simulink library "Model_DG_CHP_Plant_Simscape"  (R2022b)
settings: Solver=VariableStepAuto  StartTime=0.0  StopTime=10.0  RelTol=1e-3
undefined symbols (not defined in the file): _cos_phi, _Q, _with_const_Q, a, b, c, d, P, V
libraries: ee_lib x11, nesl_utility x11, simulink x9, fl_lib x8, sps_avr x5, spsPositiveSequencePLLDrivenLib x3, eeGeneralControl x2, slpidlib x2, spsAC1AExcitationSystemLib x1, spsST2AExcitationSystemLib x1, Sublib_InternalFunctions x1, spsPLL3phLib x1
(part 1 of 2)
settings Model: Creator=winkens  LastModifiedBy=winkens
settings SolverCC: AlgebraicLoopSolver=TrustRegion
settings DebuggingCC: UnconnectedInputMsg=warning  UnconnectedOutputMsg=warning  UnconnectedLineMsg=warning  SFMachineParentedDataDiag=warning
settings ModelReferenceCC: EnableRefExpFcnMdlSchedulingChecks=on
settings RTWCC: DLArmComputeVersion=19.05

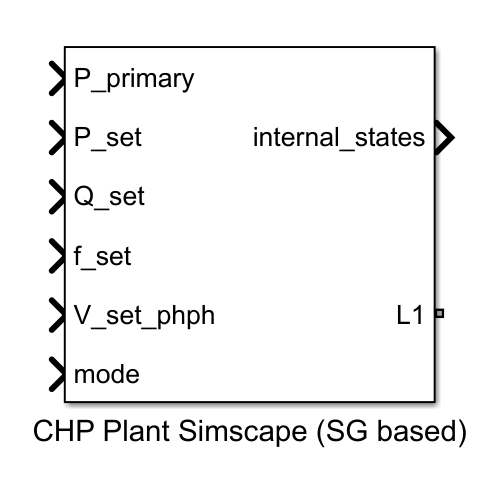
[thumbnail: Simulink's stored preview of the top-level diagram]
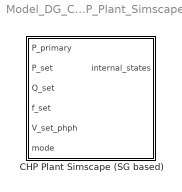
== system Model_DG_CHP_Plant_Simscape ==
  CHP Plant Simscape (SG based) : Subsystem  mask{S_n=3.2e6, V_n_phph=400, V_n_grid_phph=20e3, f_n=50, T_s=1e-4, nPolePairs=2, ReactancesSM=[3.19 0.33 0.159 1.79 0.155 0.05], X0=0.15, Ra=0.00074, TimeConstants=[0.5 0.025 0.025], K_IEEEG1simp=10, T_IEEEG1simp=[ 0.2 0 0.1 0 ], dP_maxmin_IEEEG1simp=[ 2 -2 ], exciterModel=AC1A, QCtrl=(d) Constant cos(phi), K_p_QCtrl=0.5, K_i_QCtrl=0.4, uq0ref=1.0, qmax=0.33, umax=1.04, deadband=0, p_pu=[0.1, 0.5, 0.6, 0.9, 1.0], q_pu=[0.0, 0.0, -0.05, -0.33, -0.33], p1=[0.94, 0.33], p2=[0.96, 0], p3=[1.04, 0], p4=[1.06, -0.33], cosphi_ref=1, ind_cap_Q=Inductive behavior (capacitive Q infeed), RL_Trafo_GenSide=[ 0.002 0.08 ], RL_Trafo_GridSide=[ 0.002 0.08 ], Rm=500, Lm=500, pu_X0=0.5}
      mask prompts: S_n "Nominal Apparent Power [VA]"; V_n_phph "Nominal Generator Voltage (rms, phase-to-phase) [V]"; V_n_grid_phph "Nominal Grid Voltage (rms, phase-to-phase) [V]"; f_n "Nominal Frequency [Hz]"; T_s "Sample Time [s]"; nPolePairs "Number of pole pairs"; ReactancesSM "Reactances Synchronous Machine [Xd Xd' Xd'' Xq Xq'' Xl] (pu)"; X0 "zero-sequence reactance X0 (pu)"; Ra "Stator Resistance Ra (pu)"; TimeConstants "Time Constants [Td' Td'' Tq''] (s)"; K_IEEEG1simp "Droop Gain dP/df (pu)"; T_IEEEG1simp "Time Constants [ T1 T2 T3 T4 ] (s)"; dP_maxmin_IEEEG1simp "Max. rate of change of mech. power [ dP_max dP_min ] (pu)"; exciterModel "Exciter Type"; QCtrl "Mode"; K_p_QCtrl "Q-Controller Proportional Gain"; K_i_QCtrl "Q-Controller Integral Gain"; uq0ref "U_Q0ref [pu]"; qmax "|Q_max| [pu]"; umax "U_max [pu]"; deadband "Voltage Deadband [+- %]"; p_pu "P_grid points [pu]"; q_pu "Q_grid points [pu]"; p1 "P1 [V_grid, Q_grid] [pu]"; p2 "P2 [V_grid, Q_grid] [pu]"; p3 "P3 [V_grid, Q_grid] [pu]"; p4 "P4 [V_grid, Q_grid] [pu]"; cosphi_ref "cos(phi)"; RL_Trafo_GenSide "Generator-Side-Impedance [ R L ] (pu):"; RL_Trafo_GridSide "Grid-Side-Impedance [ R L ] (pu):"; Rm "Magnetization resistance"; Lm "Magnetization inductance"; pu_X0 "zero sequence reactance"
      mask TypeOptions exciterModel: AC1A | AC4A | AC5A | DC1A | DC2A | ST1A | ST2A
      mask Callback exciterModel:
      | if strcmp(get_param(gcb,'exciterModel'),'AC1A')
      |     set_param([gcb '/SG_Control/Exciter'],'LabelModeActivechoice','AC1A');
      | 
      | elseif strcmp(get_param(gcb,'exciterModel'),'AC4A')
      |     set_param([gcb '/SG_Control/Exciter'],'LabelModeActivechoice','AC4A');
      | 
      | elseif strcmp(get_param(gcb,'exciterModel'),'AC5A')
      |     set_param([gcb '/SG_Control/Exciter'],'LabelModeActivechoice','AC5A');
      | 
      | elseif strcmp(get_param(gcb,'exciterModel'),'DC1A')
      |     set_param([gcb '/SG_Control/Exciter'],'LabelModeActivechoice','DC1A');
      | 
      | elseif strcmp(get_param(gcb,'exciterModel'),'DC2A')
      |     set_param([gcb '/SG_Control/Exciter'],'LabelModeActivechoice','DC2A');
      | 
      | elseif strcmp(get_param(gcb,'exciterModel'),'ST1A')
      |     set_param([gcb '/SG_Control/Exciter'],'LabelModeActivechoice','ST1A');
      | 
      | elseif strcmp(get_param(gcb,'exciterModel'),'ST2A')
      |     set_param([gcb '/SG_Control/Exciter'],'LabelModeActivechoice','ST2A');
      | 
      | else
      |     set_param([gcb '/SG_Control/Exciter'],'LabelModeActivechoice','DC1A');
      | 
      | end
      mask TypeOptions QCtrl: Constant Voltage (no Q-Control) | (a) Q(V)-Curve | (b) Q(P)-Curve | (c) Constant Q with Q(V)-Limitation | (d) Constant cos(phi)
      mask Callback QCtrl:
      | msk = Simulink.Mask.get(gcb);
      | if strcmp(get_param(gcb,'QCtrl'),'Constant Voltage (no Q-Control)')
      |     % no Q-Control
      |     msk.getDialogControl('paramboxVDE4110_Q_a').Visible = 'off';
      |     msk.getDialogControl('paramboxVDE4110_Q_b').Visible = 'off';
      |     msk.getDialogControl('paramboxVDE4110_Q_c').Visible = 'off';
      |     msk.getDialogControl('paramboxVDE4110_Q_d').Visible = 'off';
      |     set_param([gcb '/SG_Control/Reactive_Power_Controller'],'LabelModeActivechoice','const_V');
      | 
      | elseif strcmp(get_param(gcb,'QCtrl'),'(a) Q(V)-Curve')
      |     %(a) Q(V)
      |     msk.getDialogControl('paramboxVDE4110_Q_a').Visible = 'on';
      |     msk.getDialogControl('paramboxVDE4110_Q_b').Visible = 'off';
      |     msk.getDialogControl('paramboxVDE4110_Q_c').Visible = 'off';
      |     msk.getDialogControl('paramboxVDE4110_Q_d').Visible = 'off';
      |     set_param([gcb '/SG_Control/Reactive_Power_Controller'],'LabelModeActivechoice','(a)_Q(V)');
      | 
      | elseif strcmp(get_param(gcb,'QCtrl'),'(b) Q(P)-Curve')
      |     %(b) Q(P)
      |     msk.getDialogControl('paramboxVDE4110_Q_a').Visible = 'off';
      |     msk.getDialogControl('paramboxVDE4110_Q_b').Visible = 'on';
      |     msk.getDialogControl('paramboxVDE4110_Q_c').Visible = 'off';
      |     msk.getDialogControl('paramboxVDE4110_Q_d').Visible = 'off';
      |     set_param([gcb '/SG_Control/Reactive_Power_Controller'],'LabelModeActivechoice','(b)_Q(P)');
      | 
      | elseif strcmp(get_param(gcb,'QCtrl'),'(c) Constant Q with Q(V)-Limitation')
      |     %(c) const Q
      |     msk.getDialogControl('paramboxVDE4110_Q_a').Visible = 'off';
      |     msk.getDialogControl('paramboxVDE4110_Q_b').Visible = 'off';
      |     msk.getDialogControl('paramboxVDE4110_Q_c').Visible = 'on';
      |     msk.getDialogControl('paramboxVDE4110_Q_d').Visible = 'off';
      |     set_param([gcb '/SG_Control/Reactive_Power_Controller'],'LabelModeActivechoice','(c)_Q(V)_with_const_Q');
      | 
      | elseif strcmp(get_param(gcb,'QCtrl'),'(d) Constant cos(phi)')
      |     %(d) const cosphi
      |     msk.getDialogControl('paramboxVDE4110_Q_a').Visible = 'off';
      |     msk.getDialogControl('paramboxVDE4110_Q_b').Visible = 'off';
      |     msk.getDialogControl('paramboxVDE4110_Q_c').Visible = 'off';
      |     msk.getDialogControl('paramboxVDE4110_Q_d').Visible = 'on';
      |     set_param([gcb '/SG_Control/Reactive_Power_Controller'],'LabelModeActivechoice','(d)_cos_phi');
      | 
      | else
      |     % no Q-Control
      |     set_param([gcb '/SG_Control/Reactive_Power_Controller'],'LabelModeActivechoice','const_V');
      | 
      | end
      mask TypeOptions uq0ref: SG_Control/Reactive_Power_Controller/(a)_Q(V)/Q(V)_curve/uq0ref
      mask TypeOptions qmax: SG_Control/Reactive_Power_Controller/(a)_Q(V)/Q(V)_curve/qmax
      mask TypeOptions umax: SG_Control/Reactive_Power_Controller/(a)_Q(V)/Q(V)_curve/umax
      mask TypeOptions deadband: SG_Control/Reactive_Power_Controller/(a)_Q(V)/Q(V)_curve/deadband
      mask TypeOptions p_pu: SG_Control/Reactive_Power_Controller/(b)_Q(P)/Q(P)-curve/p_pu
      mask TypeOptions q_pu: SG_Control/Reactive_Power_Controller/(b)_Q(P)/Q(P)-curve/q_pu
      mask TypeOptions p1: SG_Control/Reactive_Power_Controller/(c)_Q(V)_with_const_Q/Q(V)_with_const_Q/p1
      mask TypeOptions p2: SG_Control/Reactive_Power_Controller/(c)_Q(V)_with_const_Q/Q(V)_with_const_Q/p2
      mask TypeOptions p3: SG_Control/Reactive_Power_Controller/(c)_Q(V)_with_const_Q/Q(V)_with_const_Q/p3
      mask TypeOptions p4: SG_Control/Reactive_Power_Controller/(c)_Q(V)_with_const_Q/Q(V)_with_const_Q/p4
      mask TypeOptions cosphi_ref: SG_Control/Reactive_Power_Controller/(d)_cos_phi/Constant_cos_phi/cosphi_ref
      mask TypeOptions ind_cap_Q: SG_Control/Reactive_Power_Controller/(d)_cos_phi/Constant_cos_phi/ind_cap_Q
      mask DialogControl DescGroupVar Prompt: CHP Plant (SG based)
      mask DialogControl DescTextVar Prompt: Combined-heat-and-power (CHP) plant using a synchronous generator (directly coupled to the grid) for electromechanical energy conversion.
      mask DialogControl Container4 Prompt: General
      mask DialogControl Container5 Prompt: Synchr. Gen.
      mask DialogControl Control2 Prompt: All Synchronous Generator Parameters are defined in a per-unit-system based on the nominal apparent power, nominal generator voltage and nominal frequency defined in general-tab.
      mask DialogControl Container11 Prompt: Parameters
      mask DialogControl Container6 Prompt: Governor
      mask DialogControl Container13 Prompt: Parameters (Simplified IEEEG1-Governor-Turbine-Model)
      mask DialogControl Container7 Prompt: Exciter
      mask DialogControl Container8 Prompt: Q-Control
      mask DialogControl Control3 Prompt: Quasi-steady state reactive power control based on German MV grid codes VDE4110. Choose constant voltage mode for no reactive power control.
      mask DialogControl Container17 Prompt: Parameters
      mask DialogControl paramboxVDE4110_Q_a Prompt: Q(V) Parameters
      mask DialogControl paramboxVDE4110_Q_b Prompt: Q(P) Parameters
      mask DialogControl paramboxVDE4110_Q_c Prompt: Constant Q with Q(V)-Limitation Parameters
      mask DialogControl paramboxVDE4110_Q_d Prompt: Constant cos(phi) Parameters
      mask DialogControl Container10 Prompt: Transformer
      mask DialogControl Control4 Prompt: Transformer parameters are defined in a per-unit-system based on the nominal power, the nominal frequency and the nominal voltages defined in tab General. The reference voltage for the impedance values depends on the respective nominal voltage level. However, magnetization resistance and inductance are based on the generator-side nominal voltage.
      mask DialogControl Container20 Prompt: Parameters

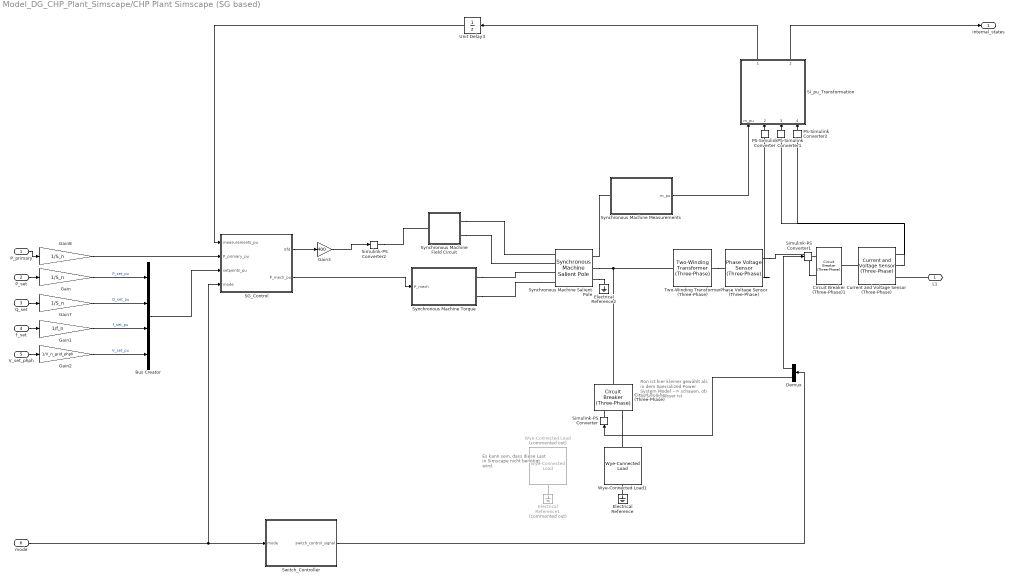
== system Model_DG_CHP_Plant_Simscape/CHP Plant Simscape (SG based) ==
  note: Ron ist hier kleiner gewählt als in dem Specialized Power System Model --> schauen, ob es so vllt besser ist
  note: Es kann sein, dass diese Last in Simscape nicht benötigt wird.
  P_primary : Inport
  P_set : Inport  Port=2
  Q_set : Inport  Port=3
  f_set : Inport  Port=4
  V_set_phph : Inport  Port=5
  mode : Inport  Port=6
  Bus Creator : BusCreator  Inputs=4
  Circuit Breaker (Three-Phase) : ee_lib/Switches & Breakers/Circuit Breaker (Three-Phase)  R_closed=0.001 Ohm  G_open=1e-6 1/Ohm  threshold=0.5 V  breaker_behavior=ee.enum.switches.breakerBehavior.zeroCrossingEnable
      settings: InternalSimscapePortConfiguration="{\"Bottom\":[],\"Left\":[{\"id\":\"vT\",\"label\":\"vT\",\"type\":\"input\"},{\"id\":\"N1\",\"label\":\"~1\",\"type\":\"foundation.electrical.three_phase\"}],\"Right\":[{\"id\":\"N2\",\"label\":\"~2\",\"type\":\"foundation.electrical.three_phase\"}],\"Top\":[]}"
  Circuit Breaker (Three-Phase)1 : ee_lib/Switches & Breakers/Circuit Breaker (Three-Phase)  R_closed=0.001 Ohm  G_open=1e-6 1/Ohm  threshold=0.5 V  breaker_behavior=ee.enum.switches.breakerBehavior.zeroCrossingEnable
      settings: InternalSimscapePortConfiguration="{\"Bottom\":[],\"Left\":[{\"id\":\"vT\",\"label\":\"vT\",\"type\":\"input\"},{\"id\":\"N1\",\"label\":\"~1\",\"type\":\"foundation.electrical.three_phase\"}],\"Right\":[{\"id\":\"N2\",\"label\":\"~2\",\"type\":\"foundation.electrical.three_phase\"}],\"Top\":[]}"
  Current and Voltage Sensor (Three-Phase) : ee_lib/Sensors & Transducers/Current and Voltage Sensor (Three-Phase)  vMeasurementType=ee.enum.vmeasurement.lg  outputUnit=ee.enum.unit.si  SRated=100e6 V*A  VRated=24e3 V  I_specify=off  I_priority=None  I=[ 0 0 0 ] A  I_nominal_specify=off  I_nominal_unit=A  I_nominal_value=1  V_specify=off  V_priority=None  V=[ 0 0 0 ] V  V_nominal_specify=off  V_nominal_unit=V  V_nominal_value=1
      settings: InternalSimscapePortConfiguration="{\"Bottom\":[],\"Left\":[{\"id\":\"N1\",\"label\":\"~1\",\"type\":\"foundation.electrical.three_phase\"}],\"Right\":[{\"id\":\"V_output\",\"label\":\"V\",\"type\":\"output\"},{\"id\":\"I_output\",\"label\":\"I\",\"type\":\"output\"},{\"id\":\"N2\",\"label\":\"~2\",\"type\":\"foundation.electrical.three_phase\"}],\"Top\":[]}"
  Demux : Demux  Outputs=2
  Electrical Reference : fl_lib/Electrical/Electrical Elements/Electrical Reference
  Electrical Reference1 : fl_lib/Electrical/Electrical Elements/Electrical Reference  Commented=on
  Electrical Reference2 : fl_lib/Electrical/Electrical Elements/Electrical Reference
  Gain : Gain  Gain=1/S_n
  Gain1 : Gain  Gain=1/f_n
  Gain2 : Gain  Gain=1/V_n_grid_phph
  Gain3 : Gain  Gain=400
  Gain7 : Gain  Gain=1/S_n
  Gain8 : Gain  Gain=1/S_n
  PS-Simulink Converter : nesl_utility/PS-Simulink Converter  PhysicalDomain=network_engine_domain  SubClassName=ps_output  LeftPortType=input  RightPortType=output  PseudoPeriodic=off  Frequencies=[]  VectorFormat=1-D array  Unit=inherit  AffineConversion=off
  PS-Simulink Converter1 : nesl_utility/PS-Simulink Converter  PhysicalDomain=network_engine_domain  SubClassName=ps_output  LeftPortType=input  RightPortType=output  PseudoPeriodic=off  Frequencies=[]  VectorFormat=1-D array  Unit=inherit  AffineConversion=off
  PS-Simulink Converter2 : nesl_utility/PS-Simulink Converter  PhysicalDomain=network_engine_domain  SubClassName=ps_output  LeftPortType=input  RightPortType=output  PseudoPeriodic=off  Frequencies=[]  VectorFormat=1-D array  Unit=inherit  AffineConversion=off
  Phase Voltage Sensor (Three-Phase) : ee_lib/Sensors & Transducers/Phase Voltage Sensor (Three-Phase)
  SG_Control : Subsystem
  SI_pu_Transformation : Subsystem
  Simulink-PS Converter : nesl_utility/Simulink-PS Converter  PhysicalDomain=network_engine_domain  SubClassName=ps_input  LeftPortType=input  RightPortType=output  PseudoPeriodic=off  Frequencies=[]  NoiseDistribution=none  NoiseParameters=[]  Unit=1  AffineConversion=off  FilteringAndDerivatives=provide  SimscapeFilterOrder=1  InputFilterTimeConstant=0.001  UdotUserProvided=0
  Simulink-PS Converter1 : nesl_utility/Simulink-PS Converter  PhysicalDomain=network_engine_domain  SubClassName=ps_input  LeftPortType=input  RightPortType=output  PseudoPeriodic=off  Frequencies=[]  NoiseDistribution=none  NoiseParameters=[]  Unit=1  AffineConversion=off  FilteringAndDerivatives=provide  SimscapeFilterOrder=1  InputFilterTimeConstant=0.001  UdotUserProvided=0
  Simulink-PS Converter2 : nesl_utility/Simulink-PS Converter  PhysicalDomain=network_engine_domain  SubClassName=ps_input  LeftPortType=input  RightPortType=output  PseudoPeriodic=off  Frequencies=[]  NoiseDistribution=none  NoiseParameters=[]  Unit=1  AffineConversion=off  FilteringAndDerivatives=provide  SimscapeFilterOrder=1  InputFilterTimeConstant=0.001  UdotUserProvided=0
  Switch_Controller : Subsystem
  Synchronous Machine Salient Pole : ee_lib/Electromechanical/Synchronous/Synchronous Machine Salient Pole  port_option=ee.enum.threePhasePort.composite  SRated=S_n V*A  VRated=V_n_phph V  FRated=f_n Hz  nPolePairs=2  param_option=ee.enum.sm.parameterization.standard  fieldCircuitParameterization_option=ee.enum.sm.fieldparameterization.current  baseEfd=400 V  baseIfd=22 A  zero_sequence=ee.enum.park.zerosequence.include  axes_param=ee.enum.rotorangle.daxis  Ladu=0.9  Laqu=0.55  L0=0.15  Ll=0.15  Ra=Ra  Lfd=0.2571  Rfd=0.0006  L1d=0.2  R1d=0.0354  L1q=0.2567  R1q=0.0428  Xl=ReactancesSM(6)  Xd=ReactancesSM(1)  Xq=ReactancesSM(4)  X0=X0  Xdd=ReactancesSM(2)  Xddd=ReactancesSM(3)  Xqdd=ReactancesSM(5)  d_option=ee.enum.circuit.short  Td0d=5.25 s  Tdd=TimeConstants(1) s  Td0dd=0.03 s  Tddd=TimeConstants(2) s  q_option=ee.enum.circuit.short  Tq0dd=0.05 s  Tqdd=TimeConstants(3) s  saturation_option=ee.enum.saturation.exclude  saturation_ifd=[0, .48, .76, 1.38, 1.79]  saturation_Vag=[0, .43, .59, .71, .76]  initialization_option=ee.enum.sm.initialization.electrical  source_type=ee.enum.sm.load_flow_source_type.Swing  Vmag0=V_n_phph V  Vang0=0 deg  Pt0=1.2e6 V*A  Qt0=0.4e6 V*A  minimum_pu=0.95  phase_search_range=[-30, 30] deg  gmin=0 S  connection_option=ee.enum.Connection.wye  num_q_dampers=1  rotor_offset=-pi / 2 rad  pu_psid_specify=on  pu_psid_priority=High  pu_psid=0  pu_psid_nominal_specify=off  pu_psid_nominal_unit=1  pu_psid_nominal_value=1  pu_psiq_specify=on  pu_psiq_priority=High  pu_psiq=0  pu_psiq_nominal_specify=off  pu_psiq_nominal_unit=1  pu_psiq_nominal_value=1  pu_psifd_specify=on  pu_psifd_priority=High  pu_psifd=0  pu_psifd_nominal_specify=off  pu_psifd_nominal_unit=1  pu_psifd_nominal_value=1  pu_psi1d_specify=on  pu_psi1d_priority=High  pu_psi1d=0  pu_psi1d_nominal_specify=off  pu_psi1d_nominal_unit=1  pu_psi1d_nominal_value=1  pu_psi1q_specify=on  pu_psi1q_priority=High  pu_psi1q=0  pu_psi1q_nominal_specify=off  pu_psi1q_nominal_unit=1  pu_psi1q_nominal_value=1  angular_position_diff_specify=on  angular_position_diff_priority=High  angular_position_diff=-pi/2/nPolePairs rad  angular_position_diff_nominal_specify=off  angular_position_diff_nominal_unit=deg  angular_position_diff_nominal_value=1  Tmeas=298.15 K  alpha=3.93e-3 1/K  stator_thermal_mass=100 J/K  rotor_thermal_mass=200 J/K  temperatureA_specify=off  temperatureA_priority=High  temperatureA=25 degC  temperatureA_nominal_specify=off  temperatureA_nominal_unit=degC  temperatureA_nominal_value=1  temperatureB_specify=off  temperatureB_priority=High  temperatureB=25 degC  temperatureB_nominal_specify=off  temperatureB_nominal_unit=degC  temperatureB_nominal_value=1  temperatureC_specify=off  temperatureC_priority=High  temperatureC=25 degC  temperatureC_nominal_specify=off  temperatureC_nominal_unit=degC  temperatureC_nominal_value=1  temperatureR_specify=off  temperatureR_priority=High  temperatureR=25 degC  temperatureR_nominal_specify=off  temperatureR_nominal_unit=degC  temperatureR_nominal_value=1
      settings: InternalSimscapePortConfiguration="{\"Bottom\":[],\"Left\":[{\"id\":\"fd_p\",\"label\":\"fd+\",\"type\":\"foundation.electrical.electrical\"},{\"id\":\"fd_n\",\"label\":\"fd-\",\"type\":\"foundation.electrical.electrical\"},{\"id\":\"R\",\"label\":\"R\",\"type\":\"foundation.mechanical.rotational.rotational\"},{\"id\":\"C\",\"label\":\"C\",\"type\":\"foundation.mechanical.rotational.rotational\"}],\"Right\":[{\"id\":\"pu_output\",\"label\":\"pu\",\"type\":\"output\"},{\"id\":\"N\",\"label\":\"~\",\"type\":\"foundation.electrical.three_phase\"},{\"id\":\"n\",\"label\":\"n\",\"type\":\"foundation.electrical.electrical\"}],\"Top\":[]}"
  Synchronous Machine Field Circuit : Subsystem
  Synchronous Machine Measurements : Subsystem
  Synchronous Machine Torque : Subsystem
  Two-Winding Transformer (Three-Phase) : ee_lib/Passive/Transformers/Two-Winding Transformer (Three-Phase)  SRated=S_n V*A  FRated=f_n Hz  Winding1Connection=ee.enum.windingconnection.Yg  VRated1=V_n_phph V  Winding2Connection=ee.enum.windingconnection.delta11  VRated2=V_n_grid_phph V  CoreType=ee.enum.coretype.threelimb  pu_Rw1=RL_Trafo_GenSide(1)  pu_Rw2=RL_Trafo_GridSide(1)  leakage_reactance_option=ee.enum.transformer_leakage.include  pu_Xl1=RL_Trafo_GenSide(2)  pu_Xl2=RL_Trafo_GridSide(2)  magnetizing_resistance_option=ee.enum.transformer_magnetizingResistance.include  pu_Rm=Rm  magnetizing_reactance_option=ee.enum.transformer_magnetizingReactance.include  saturation_option=ee.enum.transformer_saturation.exclude  pu_Xm=Lm  current_data=[0, .002, 1, 2]  magnetic_flux_data=[0, 1.2, 1.5, 1.51]  pu_X0=pu_X0  i1_specify=off  i1_priority=None  i1=[ 0 0 0 ] A  i1_nominal_specify=off  i1_nominal_unit=A  i1_nominal_value=1  i2_specify=off  i2_priority=None  i2=[ 0 0 0 ] A  i2_nominal_specify=off  i2_nominal_unit=A  i2_nominal_value=1  phi_specify=off  phi_priority=None  phi=[ 0 0 0 ]  phi_nominal_specify=off  phi_nominal_unit=1  phi_nominal_value=1  power_dissipated_specify=off  power_dissipated_priority=None  power_dissipated=0 W  power_dissipated_nominal_specify=off  power_dissipated_nominal_unit=W  power_dissipated_nominal_value=1
      settings: InternalSimscapePortConfiguration="{\"Bottom\":[],\"Left\":[{\"id\":\"N1\",\"label\":\"~1\",\"type\":\"foundation.electrical.three_phase\"}],\"Right\":[{\"id\":\"N2\",\"label\":\"~2\",\"type\":\"foundation.electrical.three_phase\"}],\"Top\":[]}"
  Unit Delay3 : UnitDelay  SampleTime=-1  HasFrameUpgradeWarning=on
  Wye-Connected Load : ee_lib/Passive/RLC Assemblies/Wye-Connected Load  Commented=on  parameterization=2  component_structure=1  component_structure_PQ=1  R=1 Ohm  L=1e-3 H  C=1e-6 F  VRated=V_n_phph V  FRated=60 Hz  P=0.001*S_n W  Qpos=1e2 V*A  Qneg=-1e2 V*A  R_parasitic=1e-6 Ohm  G_parasitic=1e-6 1/Ohm  R_parasitic_PQ=1e-6 Ohm  G_parasitic_PQ=1e-6 1/Ohm  Vmag0=24e3 V  Vang0=0 deg  Freq0=60 Hz  IL_specify=on  IL_priority=High  IL=[0, 0, 0] A  IL_nominal_specify=off  IL_nominal_unit=A  IL_nominal_value=1  VC_specify=on  VC_priority=High  VC=[0, 0, 0] V  VC_nominal_specify=off  VC_nominal_unit=V  VC_nominal_value=1
  Wye-Connected Load1 : ee_lib/Passive/RLC Assemblies/Wye-Connected Load  parameterization=2  component_structure=1  component_structure_PQ=1  R=1 Ohm  L=1e-3 H  C=1e-6 F  VRated=V_n_phph V  FRated=60 Hz  P=0.2*S_n W  Qpos=1e2 V*A  Qneg=-1e2 V*A  R_parasitic=1e-6 Ohm  G_parasitic=1e-6 1/Ohm  R_parasitic_PQ=1e-6 Ohm  G_parasitic_PQ=1e-6 1/Ohm  Vmag0=24e3 V  Vang0=0 deg  Freq0=60 Hz  IL_specify=on  IL_priority=High  IL=[0, 0, 0] A  IL_nominal_specify=off  IL_nominal_unit=A  IL_nominal_value=1  VC_specify=on  VC_priority=High  VC=[0, 0, 0] V  VC_nominal_specify=off  VC_nominal_unit=V  VC_nominal_value=1
  L1 : PMIOPort  Side=Right
  internal_states : Outport
  wires:
  V_set_phph/1 -> Gain2/1
  P_set/1 -> Gain/1
  f_set/1 -> Gain1/1
  SI_pu_Transformation/2(measurements_SI) -> internal_states/1
  SI_pu_Transformation/1(measurements_pu) -> Unit Delay3/1
  Q_set/1 -> Gain7/1
  P_primary/1 -> Gain8/1
  Gain/1 -> Bus Creator/1  "P_set_pu"
  Gain7/1 -> Bus Creator/2  "Q_set_pu"
  Gain1/1 -> Bus Creator/3  "f_set_pu"
  Gain2/1 -> Bus Creator/4  "V_set_pu"
  Switch_Controller/1(switch_control_signal) -> Demux/1
  Demux/2 -> Simulink-PS Converter/1
  PS-Simulink Converter/1 -> SI_pu_Transformation/2(V_breaker_SI)
  Demux/1 -> Simulink-PS Converter1/1
  PS-Simulink Converter1/1 -> SI_pu_Transformation/3(V_grid_SI)
  PS-Simulink Converter2/1 -> SI_pu_Transformation/4(I_grid_SI)
  Gain8/1 -> SG_Control/2(P_primary_pu)
  mode/1 -> SG_Control/4(mode), Switch_Controller/1(mode)
  Bus Creator/1 -> SG_Control/3(setpoints_pu)
  Unit Delay3/1 -> SG_Control/1(measurements_pu)
  Synchronous Machine Measurements/1(m_pu) -> SI_pu_Transformation/1(m_pu)
  SG_Control/2(P_mech_pu) -> Synchronous Machine Torque/1(P_mech)
  Gain3/1 -> Simulink-PS Converter2/1
  SG_Control/1(Efd) -> Gain3/1
  connections:
  Synchronous Machine Salient Pole/RConn2 -- Two-Winding Transformer (Three-Phase)/LConn1 -- Circuit Breaker (Three-Phase)/RConn1
  Circuit Breaker (Three-Phase)/LConn2 -- Wye-Connected Load1/LConn1
  Simulink-PS Converter/RConn1 -- Circuit Breaker (Three-Phase)/LConn1
  Electrical Reference/LConn1 -- Wye-Connected Load1/RConn1
  Electrical Reference1/LConn1 -- Wye-Connected Load/RConn1
  Two-Winding Transformer (Three-Phase)/RConn1 -- Phase Voltage Sensor (Three-Phase)/LConn1
  Phase Voltage Sensor (Three-Phase)/RConn1 -- PS-Simulink Converter/LConn1
  Phase Voltage Sensor (Three-Phase)/RConn2 -- Circuit Breaker (Three-Phase)1/LConn2
  Simulink-PS Converter1/RConn1 -- Circuit Breaker (Three-Phase)1/LConn1
  Current and Voltage Sensor (Three-Phase)/LConn1 -- Circuit Breaker (Three-Phase)1/RConn1
  Current and Voltage Sensor (Three-Phase)/RConn2 -- PS-Simulink Converter2/LConn1
  L1/RConn1 -- Current and Voltage Sensor (Three-Phase)/RConn3
  Synchronous Machine Salient Pole/RConn3 -- Electrical Reference2/LConn1
  PS-Simulink Converter1/LConn1 -- Current and Voltage Sensor (Three-Phase)/RConn1
  Simulink-PS Converter2/RConn1 -- Synchronous Machine Field Circuit/LConn1
  Synchronous Machine Field Circuit/RConn1 -- Synchronous Machine Salient Pole/LConn1
  Synchronous Machine Field Circuit/RConn2 -- Synchronous Machine Salient Pole/LConn2
  Synchronous Machine Salient Pole/RConn1 -- Synchronous Machine Measurements/LConn1
  Synchronous Machine Torque/RConn1 -- Synchronous Machine Salient Pole/LConn3
  Synchronous Machine Torque/RConn2 -- Synchronous Machine Salient Pole/LConn4

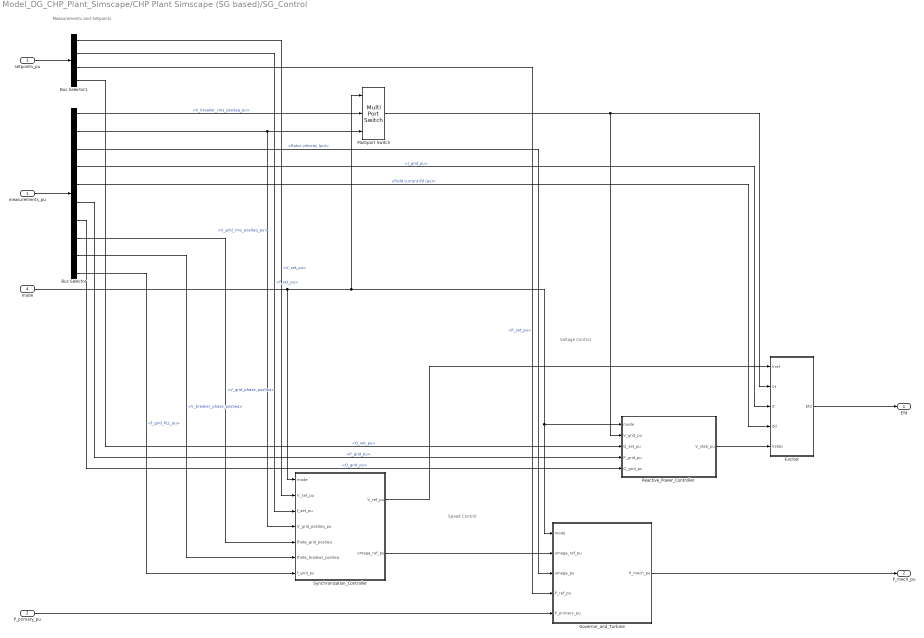
== system Model_DG_CHP_Plant_Simscape/CHP Plant Simscape (SG based)/SG_Control ==
  note: Speed Control
  note: Voltage Control
  note: Measurements and Setpoints
  measurements_pu : Inport
  P_primary_pu : Inport  Port=2
  setpoints_pu : Inport  Port=3
  mode : Inport  Port=4
  Bus Selector : BusSelector  OutputSignals=electrical_pu.V_breaker_rms_posSeq_pu,electrical_pu.V_grid_rms_posSeq_pu,SG_pu.Rotor velocity (pu),electrical_pu.I_grid_pu,SG_pu.Field current Ifd (pu),electrical_pu.P_grid_pu,electrical_pu.Q_grid_pu,electrical_pu.V_grid_phase_posSeq,electrical_pu.V_breaker_phase_posSeq,electrical_pu.f_grid_PLL_pu
  Bus Selector1 : BusSelector  OutputSignals=V_set_pu,f_set_pu,P_set_pu,Q_set_pu
  Exciter : Subsystem  Variant=on  VariantControlMode=label  LabelModeActiveChoice=AC1A
      settings: AttributesFormatString=%<BlockChoice>
  Governor_and_Turbine : Subsystem  Variant=on  VariantControlMode=label  LabelModeActiveChoice=IEEEG1_simplified
  Multiport Switch : MultiPortSwitch  Inputs=2  DiagnosticForDefault=None  SaturateOnIntegerOverflow=off  InputSameDT=off
  Reactive_Power_Controller : Subsystem  Variant=on  VariantControlMode=label  LabelModeActiveChoice=(d)_cos_phi
  Synchronization_Controller : Subsystem
  Efd : Outport
  P_mech_pu : Outport  Port=2
  wires:
  Exciter/1(Efd) -> Efd/1
  Governor_and_Turbine/1(P_mech_pu) -> P_mech_pu/1
  Reactive_Power_Controller/1(V_stab_pu) -> Exciter/5(Vstab)
  measurements_pu/1 -> Bus Selector/1
  setpoints_pu/1 -> Bus Selector1/1
  Bus Selector1/3 -> Governor_and_Turbine/4(P_ref_pu)  "<P_set_pu>"
  Bus Selector/3 -> Governor_and_Turbine/3(omega_pu)  "<Rotor velocity (pu)>"
  P_primary_pu/1 -> Governor_and_Turbine/5(P_primary_pu)
  Multiport Switch/1 -> Reactive_Power_Controller/2(V_grid_pu), Exciter/2(Vt)
  Bus Selector/4 -> Exciter/3(It)  "<I_grid_pu>"
  Bus Selector/5 -> Exciter/4(Ifd)  "<Field current Ifd (pu)>"
  mode/1 -> Multiport Switch/1, Governor_and_Turbine/1(mode), Reactive_Power_Controller/1(mode), Synchronization_Controller/1(mode)
  Bus Selector1/4 -> Reactive_Power_Controller/3(Q_set_pu)  "<Q_set_pu>"
  Bus Selector/2 -> Synchronization_Controller/4(V_grid_posSeq_pu), Multiport Switch/3  "<V_grid_rms_posSeq_pu>"
  Bus Selector/1 -> Multiport Switch/2  "<V_breaker_rms_posSeq_pu>"
  Bus Selector/6 -> Reactive_Power_Controller/4(P_grid_pu)  "<P_grid_pu>"
  Bus Selector/7 -> Reactive_Power_Controller/5(Q_grid_pu)  "<Q_grid_pu>"
  Synchronization_Controller/2(omega_ref_pu) -> Governor_and_Turbine/2(omega_ref_pu)
  Synchronization_Controller/1(V_ref_pu) -> Exciter/1(Vref)
  Bus Selector1/1 -> Synchronization_Controller/2(V_set_pu)  "<V_set_pu>"
  Bus Selector1/2 -> Synchronization_Controller/3(f_set_pu)  "<f_set_pu>"
  Bus Selector/8 -> Synchronization_Controller/5(theta_grid_posSeq)  "<V_grid_phase_posSeq>"
  Bus Selector/9 -> Synchronization_Controller/6(theta_breaker_posSeq)  "<V_breaker_phase_posSeq>"
  Bus Selector/10 -> Synchronization_Controller/7(f_grid_pu)  "<f_grid_PLL_pu>"

== system Model_DG_CHP_Plant_Simscape/CHP Plant Simscape (SG based)/SI_pu_Transformation ==
  m_pu : Inport
  V_breaker_SI : Inport  Port=2
  V_grid_SI : Inport  Port=3
  I_grid_SI : Inport  Port=4
  Bus Creator : BusCreator  Inputs=11
  Bus Creator1 : BusCreator  Inputs=2
  Bus Creator2 : BusCreator  Inputs=2
  Electrical_Measurements_To_pu : Subsystem
  Positive_Sequence_Calculation : Subsystem
  SG_Measurements_To_SI : Subsystem
  measurements_pu : Outport
  measurements_SI : Outport  Port=2
  wires:
  m_pu/1 -> Bus Creator2/1, SG_Measurements_To_SI/1(m_pu)  "SG_pu"
  V_breaker_SI/1 -> Positive_Sequence_Calculation/2(V_breaker_abc), Bus Creator/1  "V_breaker_SI"
  V_grid_SI/1 -> Positive_Sequence_Calculation/1(V_grid_abc), Bus Creator/2  "V_grid_SI"
  I_grid_SI/1 -> Positive_Sequence_Calculation/3(I_grid_abc), Bus Creator/3  "I_grid_SI"
  Bus Creator/1 -> Bus Creator1/2, Electrical_Measurements_To_pu/1(el_SI)  "electrical_SI"
  Bus Creator1/1 -> measurements_SI/1
  Bus Creator2/1 -> measurements_pu/1
  Electrical_Measurements_To_pu/1(el_pu) -> Bus Creator2/2  "electrical_pu"
  SG_Measurements_To_SI/1(m_SI) -> Bus Creator1/1  "SG_SI"
  Positive_Sequence_Calculation/1(P_grid_SI) -> Bus Creator/4  "P_grid_SI"
  Positive_Sequence_Calculation/2(Q_grid_SI) -> Bus Creator/5  "Q_grid_SI"
  Positive_Sequence_Calculation/3(V_grid_rms_posSeq_SI) -> Bus Creator/6  "V_grid_rms_posSeq_SI"
  Positive_Sequence_Calculation/4(I_grid_rms_posSeq_SI) -> Bus Creator/7  "I_grid_rms_posSeq_SI"
  Positive_Sequence_Calculation/5(V_breaker_rms_posSeq_SI) -> Bus Creator/8  "V_breaker_rms_posSeq_SI"
  Positive_Sequence_Calculation/6(V_grid_phase_posSeq_SI) -> Bus Creator/9  "V_grid_phase_posSeq"
  Positive_Sequence_Calculation/7(V_breaker_phase_posSeq_SI) -> Bus Creator/10  "V_breaker_phase_posSeq"
  Positive_Sequence_Calculation/8(f_grid_PLL_SI) -> Bus Creator/11  "f_grid_PLL_SI"

== system Model_DG_CHP_Plant_Simscape/CHP Plant Simscape (SG based)/Switch_Controller ==
  note: Blackstart
  note: Synchronization
  note: Grid Parallel Operation
  mode : Inport
  Constant{,1..3} (4 alike) : Constant  Value=0
  Constant4 : Constant
  Constant5 : Constant
  Multiport Switch : MultiPortSwitch  DataPortOrder=Zero-based contiguous  zeroidx=on  SaturateOnIntegerOverflow=off  InputSameDT=off
  Mux : Mux  Inputs=2
  Mux1 : Mux  Inputs=2
  Mux2 : Mux  Inputs=2
  switch_control_signal : Outport
  wires:
  mode/1 -> Multiport Switch/1
  Multiport Switch/1 -> switch_control_signal/1
  Mux/1 -> Multiport Switch/2
  Mux2/1 -> Multiport Switch/4
  Mux1/1 -> Multiport Switch/3
  Constant/1 -> Mux/1
  Constant1/1 -> Mux/2
  Constant2/1 -> Mux2/1
  Constant3/1 -> Mux1/2
  Constant4/1 -> Mux1/1
  Constant5/1 -> Mux2/2

== system Model_DG_CHP_Plant_Simscape/CHP Plant Simscape (SG based)/Synchronous Machine Field Circuit ==
  Controlled Voltage Source : fl_lib/Electrical/Electrical Sources/Controlled Voltage Source
  Electrical Reference2 : fl_lib/Electrical/Electrical Elements/Electrical Reference
  Efd : PMIOPort  Side=Left
  fd+ : PMIOPort  Port=2  Side=Right
  fd- : PMIOPort  Port=3  Side=Right
  connections:
  Efd/RConn1 -- Controlled Voltage Source/RConn1
  Controlled Voltage Source/LConn1 -- fd+/RConn1
  Controlled Voltage Source/RConn2 -- Electrical Reference2/LConn1 -- fd-/RConn1

== system Model_DG_CHP_Plant_Simscape/CHP Plant Simscape (SG based)/Synchronous Machine Measurements ==
  Bus Creator1 : BusCreator  Inputs=2
  PS-Simulink Converter4 : nesl_utility/PS-Simulink Converter  PhysicalDomain=network_engine_domain  SubClassName=ps_output  LeftPortType=input  RightPortType=output  PseudoPeriodic=off  Frequencies=[]  VectorFormat=1-D array  Unit=inherit  AffineConversion=off
  PS-Simulink Converter5 : nesl_utility/PS-Simulink Converter  PhysicalDomain=network_engine_domain  SubClassName=ps_output  LeftPortType=input  RightPortType=output  PseudoPeriodic=off  Frequencies=[]  VectorFormat=1-D array  Unit=inherit  AffineConversion=off
  Synchronous Machine Measurement : ee_lib/Electromechanical/Synchronous/Synchronous Machine Measurement  output_idx=2
      settings: InternalSimscapePortConfiguration="{\"Bottom\":[],\"Left\":[{\"id\":\"pu_input\",\"label\":\"pu\",\"type\":\"input\"}],\"Right\":[{\"id\":\"pu_output\",\"label\":\"o\",\"type\":\"output\"}],\"Top\":[]}"
  Synchronous Machine Measurement1 : ee_lib/Electromechanical/Synchronous/Synchronous Machine Measurement  output_idx=4
      settings: InternalSimscapePortConfiguration="{\"Bottom\":[],\"Left\":[{\"id\":\"pu_input\",\"label\":\"pu\",\"type\":\"input\"}],\"Right\":[{\"id\":\"pu_output\",\"label\":\"o\",\"type\":\"output\"}],\"Top\":[]}"
  pu : PMIOPort  Side=Left
  m_pu : Outport
  wires:
  PS-Simulink Converter4/1 -> Bus Creator1/1  "Field current Ifd (pu)"
  PS-Simulink Converter5/1 -> Bus Creator1/2  "Rotor velocity (pu)"
  Bus Creator1/1 -> m_pu/1
  connections:
  Synchronous Machine Measurement/LConn1 -- Synchronous Machine Measurement1/LConn1 -- pu/RConn1
  Synchronous Machine Measurement/RConn1 -- PS-Simulink Converter4/LConn1
  Synchronous Machine Measurement1/RConn1 -- PS-Simulink Converter5/LConn1

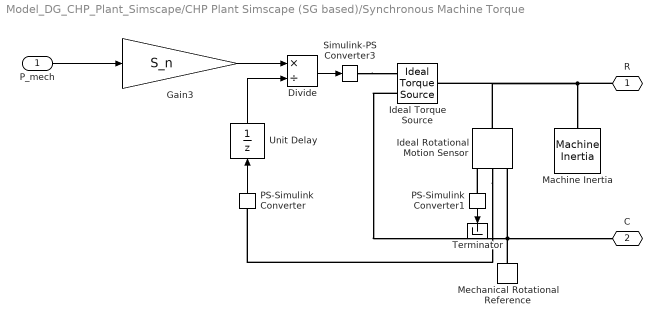
== system Model_DG_CHP_Plant_Simscape/CHP Plant Simscape (SG based)/Synchronous Machine Torque ==
  P_mech : Inport
  Divide : Product  Inputs=*/
  Gain3 : Gain  Gain=S_n
  Ideal Rotational Motion Sensor : fl_lib/Mechanical/Mechanical Sensors/Ideal Rotational Motion Sensor  reference=foundation.enum.MeasurementReference.difference  acceleration_port=false  velocity_port=true  position_port=true  wrap_angle=simscape.enum.onoff.off  offset=0 rad
  Ideal Torque Source : fl_lib/Mechanical/Mechanical Sources/Ideal Torque Source
  Machine Inertia : ee_lib/Electromechanical/Mechanical/Machine Inertia  SRated=S_n V*A  FRated=f_n Hz  nPolePairs=nPolePairs  inertia_option=2  J=27548 kg*m^2  H=0.02 s*W/V/A  damper_option=2  D=39.0509 N*m/(rad/s)  pu_D=0.01  initialization_option=2  fMechanical0=60 Hz  fElectrical0=f_n Hz
      settings: InternalSimscapePortConfiguration="{\"Bottom\":[],\"Left\":[{\"id\":\"R\",\"label\":\"R\",\"type\":\"foundation.mechanical.rotational.rotational\"}],\"Right\":[],\"Top\":[]}"
  Mechanical Rotational Reference : fl_lib/Mechanical/Rotational Elements/Mechanical Rotational Reference
  PS-Simulink Converter : nesl_utility/PS-Simulink Converter  PhysicalDomain=network_engine_domain  SubClassName=ps_output  LeftPortType=input  RightPortType=output  PseudoPeriodic=off  Frequencies=[]  VectorFormat=1-D array  Unit=inherit  AffineConversion=off
  PS-Simulink Converter1 : nesl_utility/PS-Simulink Converter  PhysicalDomain=network_engine_domain  SubClassName=ps_output  LeftPortType=input  RightPortType=output  PseudoPeriodic=off  Frequencies=[]  VectorFormat=1-D array  Unit=inherit  AffineConversion=off
  Simulink-PS Converter3 : nesl_utility/Simulink-PS Converter  PhysicalDomain=network_engine_domain  SubClassName=ps_input  LeftPortType=input  RightPortType=output  PseudoPeriodic=off  Frequencies=[]  NoiseDistribution=none  NoiseParameters=[]  Unit=1  AffineConversion=off  FilteringAndDerivatives=provide  SimscapeFilterOrder=1  InputFilterTimeConstant=0.001  UdotUserProvided=0
  Terminator : Terminator
  Unit Delay : UnitDelay  InitialCondition=(2*pi*f_n)/nPolePairs  SampleTime=-1  HasFrameUpgradeWarning=on
  R : PMIOPort  Side=Right
  C : PMIOPort  Port=2  Side=Right
  wires:
  P_mech/1 -> Gain3/1
  Gain3/1 -> Divide/1
  Divide/1 -> Simulink-PS Converter3/1
  PS-Simulink Converter/1 -> Unit Delay/1
  Unit Delay/1 -> Divide/2
  PS-Simulink Converter1/1 -> Terminator/1
  connections:
  Simulink-PS Converter3/RConn1 -- Ideal Torque Source/RConn1
  R/RConn1 -- Ideal Rotational Motion Sensor/LConn1 -- Ideal Torque Source/LConn1 -- Machine Inertia/LConn1
  Mechanical Rotational Reference/LConn1 -- C/RConn1 -- Ideal Torque Source/RConn2 -- Ideal Rotational Motion Sensor/RConn1
  Ideal Rotational Motion Sensor/RConn2 -- PS-Simulink Converter/LConn1
  PS-Simulink Converter1/LConn1 -- Ideal Rotational Motion Sensor/RConn3

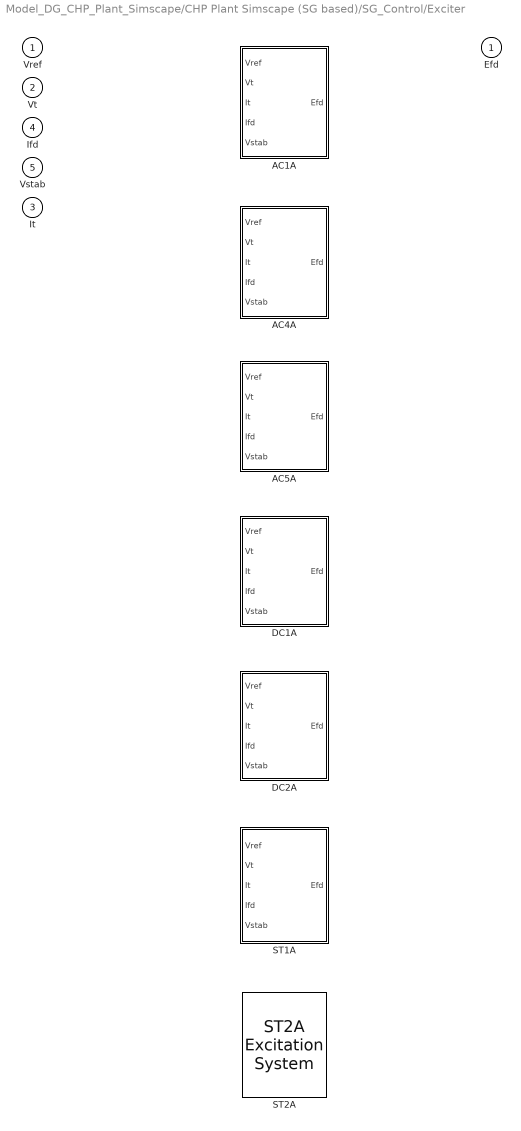
== system Model_DG_CHP_Plant_Simscape/CHP Plant Simscape (SG based)/SG_Control/Exciter ==
  Vref : Inport
  Vt : Inport  Port=2
  It : Inport  Port=3
  Ifd : Inport  Port=4
  Vstab : Inport  Port=5
  AC1A : Subsystem  VariantControl=AC1A
  AC4A : Subsystem  VariantControl=AC4A
  AC5A : Subsystem  VariantControl=AC5A
  DC1A : Subsystem  VariantControl=DC1A
  DC2A : Subsystem  VariantControl=DC2A
  ST1A : Subsystem  VariantControl=ST1A
  ST2A : spsST2AExcitationSystemLib/ST2A Excitation System  VariantControl=ST2A  Tr=20e-3  KaTa=[120 0.15]  VRminmax=[0 1.0]  KfTf=[0.05 1.0]  KeTe=[1.0 0.5]  KI=0  Kp=4.88  Xd=1.56  Kc=0.1  v0=[1,1.42734]  I0=0.2739  TsBlock=-2
  Efd : Outport  VectorParamsAs1DForOutWhenUnconnected=off

== system Model_DG_CHP_Plant_Simscape/CHP Plant Simscape (SG based)/SG_Control/Governor_and_Turbine ==
  note: 1) Add Subsystem or Model blocks as valid variant choices.
      | 2) You cannot connect blocks at this level. At simulation, connectivity is automatically
      | determined, based on the active variant and port name matching.
  mode : Inport
  omega_ref_pu : Inport  Port=2
  omega_pu : Inport  Port=3
  P_ref_pu : Inport  Port=4
  P_primary_pu : Inport  Port=5
  IEEEG1_simplified : Subsystem  VariantControl=IEEEG1_simplified
  P_mech_pu : Outport

== system Model_DG_CHP_Plant_Simscape/CHP Plant Simscape (SG based)/SG_Control/Reactive_Power_Controller ==
  note: 1) Add Subsystem or Model blocks as valid variant choices.
      | 2) You cannot connect blocks at this level. At simulation, connectivity is automatically
      | determined, based on the active variant and port name matching.
  mode : Inport
  V_grid_pu : Inport  Port=2
  Q_set_pu : Inport  Port=3
  P_grid_pu : Inport  Port=4
  Q_grid_pu : Inport  Port=5
  (a)_Q(V) : Subsystem  VariantControl=(a)_Q(V)
  (b)_Q(P) : Subsystem  VariantControl=(b)_Q(P)
  (c)_Q(V)_with_const_Q : Subsystem  VariantControl=(c)_Q(V)_with_const_Q
  (d)_cos_phi : Subsystem  VariantControl=(d)_cos_phi
  Constant_Voltage : Subsystem  VariantControl=const_V
  V_stab_pu : Outport

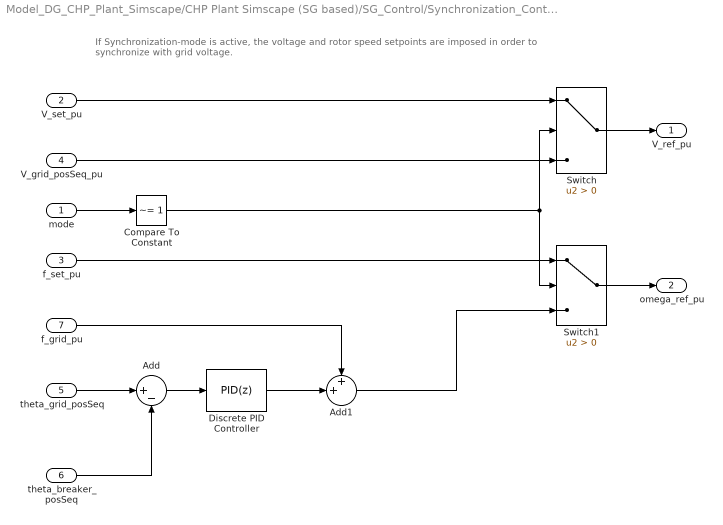
== system Model_DG_CHP_Plant_Simscape/CHP Plant Simscape (SG based)/SG_Control/Synchronization_Controller ==
  note: If Synchronization-mode is active, the voltage and rotor speed setpoints are imposed in order to synchronize with grid voltage.
  mode : Inport
  V_set_pu : Inport  Port=2
  f_set_pu : Inport  Port=3
  V_grid_posSeq_pu : Inport  Port=4
  theta_grid_posSeq : Inport  Port=5
  theta_breaker_posSeq : Inport  Port=6
  f_grid_pu : Inport  Port=7
  Add : Sum  Inputs=|+-
  Add1 : Sum  Inputs=++|
  Compare To Constant : simulink/Logic and Bit Operations/Compare To Constant  relop=~=  const=1  OutDataTypeStr=boolean
  Discrete PID Controller : slpidlib/PID Controller  Controller=PID  Form=Parallel  TimeDomain=Discrete-time  UseExternalTs=off  SampleTime=-1  IntegratorMethod=Forward Euler  FilterMethod=Forward Euler  ControllerParametersSource=internal  P=0.01  I=0.01  UseKiTs=off  D=0.01  N=100  UseFilter=on  TunerSelectOption=Transfer Function Based (PID Tuner App)  InitialConditionSource=internal  InitialConditionForIntegrator=0  InitialConditionForFilter=0  DifferentiatorICPrevScaledInput=0  ExternalReset=none  TrackingMode=off  Kt=1  LimitOutput=on  SatLimitsSource=internal  UpperSaturationLimit=0.005  LowerSaturationLimit=-0.005  LinearizeAsGain=off  AntiWindupMode=clamping  Kb=1  LimitIntegrator=off  UpperIntegratorSaturationLimit=inf  LowerIntegratorSaturationLimit=-inf  POutMin=[]  POutMax=[]  IOutMin=[]  IOutMax=[]  DOutMin=[]  DOutMax=[]  NOutMin=[]  NOutMax=[]  SumOutMin=[]  SumOutMax=[]  SaturationOutMin=[]  SaturationOutMax=[]  PParamMin=[]  PParamMax=[]  IParamMin=[]  IParamMax=[]  DParamMin=[]  DParamMax=[]  NParamMin=[]  NParamMax=[]  KbParamMin=[]  KbParamMax=[]  KtParamMin=[]  KtParamMax=[]  KbOutMin=[]  KbOutMax=[]  KtOutMin=[]  KtOutMax=[]  IntegratorOutMin=[]  IntegratorOutMax=[]  FilterOutMin=[]  FilterOutMax=[]  SumI1OutMin=[]  SumI1OutMax=[]  SumI2OutMin=[]  SumI2OutMax=[]  SumI3OutMin=[]  SumI3OutMax=[]  SumI4OutMin=[]  SumI4OutMax=[]  SumDOutMin=[]  SumDOutMax=[]  DifferentiatorOutMin=[]  DifferentiatorOutMax=[]  FilterDiffOutCoefMin=[]  FilterDiffOutCoefMax=[]  ReciprocalOutMin=[]  ReciprocalOutMax=[]  SumDenOutMin=[]  SumDenOutMax=[]  SumNumOutMin=[]  SumNumOutMax=[]  DivideOutMin=[]  DivideOutMax=[]  UdiffTsProdOutMin=[]  UdiffTsProdOutMax=[]  NTsProdOutMin=[]  NTsProdOutMax=[]  UintegralTsProdOutMin=[]  UintegralTsProdOutMax=[]  UngainTsProdOutMin=[]  UngainTsProdOutMax=[]  ClampingZeroOutDataTypeStr=Inherit: Inherit via back propagation  ClampingZeroOutMin=[]  ClampingZeroOutMax=[]  FilterDenConstantOutDataTypeStr=Inherit: Inherit via back propagation  FilterDenConstantOutMin=[]  FilterDenConstantOutMax=[]  PCopyOutDataTypeStr=Inherit: Inherit via back propagation  PCopyOutMin=[]  PCopyOutMax=[]  NCopyOutDataTypeStr=Inherit: Inherit via back propagation  NCopyOutMin=[]  NCopyOutMax=[]  IntegratorContinuousStateAttributes=''  IntegratorStateMustResolveToSignalObject=off  IntegratorRTWStateStorageClass=Auto  FilterContinuousStateAttributes=''  FilterStateMustResolveToSignalObject=off  FilterRTWStateStorageClass=Auto  ParallelPVariant=InternalParameters  IdealPVariant=Disabled  IVariant=InternalParameters  DVariant=InternalParameters  IntegratorVariant=Discrete  SatVariant=Enabled  AWVariant=DiscClampingParallel  PCopyVariant=Disabled  TRVariant=Disabled  FdbkBlocksVariant=Forward  IdealPFdbkVariant=Disabled  SatFdbkVariant=Disabled  DerivativeFilterVariant=ForwardEulerFilter  NVariant=InternalParameters  NCopyVariant=Disabled  FilterICVariant=InternalICsFilter  IntegratorICVariant=InternalICs  ExternalResetVariant=Disabled  TRSumVariant=Passthrough  SumFdbkVariant=Disabled  SumVariant=Sum_PID  TsampFilterVariant=InternalTs  TsampNgainVariant=Passthrough  TsampIntegralVariant=Passthrough  ExternalSaturationOutDataTypeStr=Inherit: Same as second input
  Switch : Switch  Criteria=u2 > Threshold  SaturateOnIntegerOverflow=off  InputSameDT=off
  Switch1 : Switch  Criteria=u2 > Threshold  SaturateOnIntegerOverflow=off  InputSameDT=off
  V_ref_pu : Outport
  omega_ref_pu : Outport  Port=2
  wires:
  mode/1 -> Compare To Constant/1
  Switch/1 -> V_ref_pu/1
  Switch1/1 -> omega_ref_pu/1
  Compare To Constant/1 -> Switch/2, Switch1/2
  f_set_pu/1 -> Switch1/1
  V_set_pu/1 -> Switch/1
  V_grid_posSeq_pu/1 -> Switch/3
  theta_grid_posSeq/1 -> Add/1
  theta_breaker_posSeq/1 -> Add/2
  Add/1 -> Discrete PID Controller/1
  Discrete PID Controller/1 -> Add1/2
  Add1/1 -> Switch1/3
  f_grid_pu/1 -> Add1/1

== system Model_DG_CHP_Plant_Simscape/CHP Plant Simscape (SG based)/SI_pu_Transformation/Electrical_Measurements_To_pu ==
  el_SI : Inport
  Bus Creator : BusCreator  Inputs=11
  Bus Selector : BusSelector  OutputSignals=V_breaker_SI,V_grid_SI,I_grid_SI,P_grid_SI,Q_grid_SI,V_grid_rms_posSeq_SI,I_grid_rms_posSeq_SI,V_breaker_rms_posSeq_SI,V_grid_phase_posSeq,V_breaker_phase_posSeq,f_grid_PLL_SI
  Gain{,1,5,7} (4 alike) : Gain  Gain=sqrt(3)/V_n_grid_phph
  Gain2 : Gain  Gain=(sqrt(3)*V_n_grid_phph) / S_n
  Gain3 : Gain  Gain=1/S_n
  Gain4 : Gain  Gain=1/S_n
  Gain6 : Gain  Gain=(sqrt(3)*V_n_grid_phph) / S_n
  Gain8 : Gain  Gain=1/f_n
  el_pu : Outport
  wires:
  el_SI/1 -> Bus Selector/1
  Bus Selector/1 -> Gain/1  "<V_breaker_SI>"
  Bus Selector/2 -> Gain1/1  "<V_grid_SI>"
  Bus Selector/3 -> Gain2/1  "<I_grid_SI>"
  Gain/1 -> Bus Creator/1  "V_breaker_pu"
  Gain1/1 -> Bus Creator/2  "V_grid_pu"
  Gain2/1 -> Bus Creator/3  "I_grid_pu"
  Bus Creator/1 -> el_pu/1
  Bus Selector/4 -> Gain3/1  "<P_grid_SI>"
  Gain3/1 -> Bus Creator/4  "P_grid_pu"
  Bus Selector/5 -> Gain4/1  "<Q_grid_SI>"
  Gain4/1 -> Bus Creator/5  "Q_grid_pu"
  Bus Selector/6 -> Gain5/1  "<V_grid_rms_posSeq_SI>"
  Gain5/1 -> Bus Creator/6  "V_grid_rms_posSeq_pu"
  Bus Selector/7 -> Gain6/1  "<I_grid_rms_posSeq_SI>"
  Gain6/1 -> Bus Creator/7  "I_grid_rms_posSeq_pu"
  Bus Selector/8 -> Gain7/1  "<V_breaker_rms_posSeq_SI>"
  Gain7/1 -> Bus Creator/8  "V_breaker_rms_posSeq_pu"
  Bus Selector/9 -> Bus Creator/9  "<V_grid_phase_posSeq>"
  Bus Selector/10 -> Bus Creator/10  "<V_breaker_phase_posSeq>"
  Bus Selector/11 -> Gain8/1  "<f_grid_PLL_SI>"
  Gain8/1 -> Bus Creator/11  "f_grid_PLL_pu"

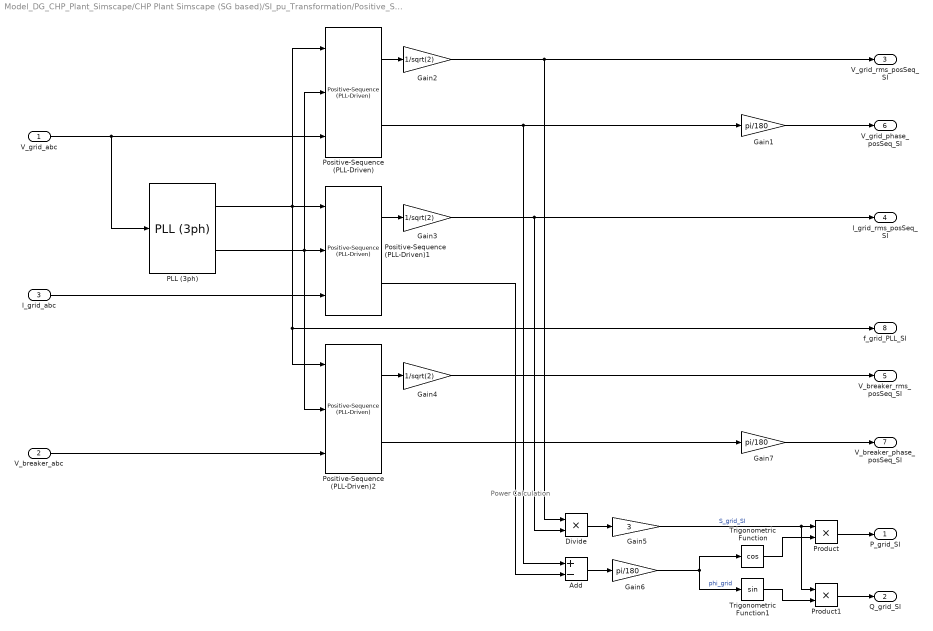
== system Model_DG_CHP_Plant_Simscape/CHP Plant Simscape (SG based)/SI_pu_Transformation/Positive_Sequence_Calculation ==
  note: Power Calculation
  V_grid_abc : Inport
  V_breaker_abc : Inport  Port=2
  I_grid_abc : Inport  Port=3
  Add : Sum  Inputs=+-
  Divide : Product  Inputs=**
  Gain1 : Gain  Gain=pi/180
  Gain2 : Gain  Gain=1/sqrt(2)
  Gain3 : Gain  Gain=1/sqrt(2)
  Gain4 : Gain  Gain=1/sqrt(2)
  Gain5 : Gain  Gain=3
  Gain6 : Gain  Gain=pi/180
  Gain7 : Gain  Gain=pi/180
  PLL (3ph) : spsPLL3phLib/PLL (3ph)  Fmin=35  Par_Init=[0, 50]  ParK=[180, 3200, 1]  TcD=1e-4  MaxRateChangeFreq=12  FilterCutOffFreq=25  Ts=1e-4  AGC=on
  Positive-Sequence (PLL-Driven) : spsPositiveSequencePLLDrivenLib/Positive-Sequence (PLL-Driven)  Finit=50  Fmin=35  InInit=[0, 0]  Ts=T_s
  Positive-Sequence (PLL-Driven)1 : spsPositiveSequencePLLDrivenLib/Positive-Sequence (PLL-Driven)  Finit=50  Fmin=35  InInit=[0, 0]  Ts=T_s
  Positive-Sequence (PLL-Driven)2 : spsPositiveSequencePLLDrivenLib/Positive-Sequence (PLL-Driven)  Finit=50  Fmin=35  InInit=[0, 0]  Ts=T_s
  Product : Product
  Product1 : Product
  Trigonometric Function : Trigonometry  Operator=cos
  Trigonometric Function1 : Trigonometry
  P_grid_SI : Outport
  Q_grid_SI : Outport  Port=2
  V_grid_rms_posSeq_SI : Outport  Port=3
  I_grid_rms_posSeq_SI : Outport  Port=4
  V_breaker_rms_posSeq_SI : Outport  Port=5
  V_grid_phase_posSeq_SI : Outport  Port=6
  V_breaker_phase_posSeq_SI : Outport  Port=7
  f_grid_PLL_SI : Outport  Port=8
  wires:
  V_grid_abc/1 -> PLL (3ph)/1, Positive-Sequence (PLL-Driven)/3
  I_grid_abc/1 -> Positive-Sequence (PLL-Driven)1/3
  V_breaker_abc/1 -> Positive-Sequence (PLL-Driven)2/3
  Positive-Sequence (PLL-Driven)2/1 -> Gain4/1
  Positive-Sequence (PLL-Driven)1/1 -> Gain3/1
  Positive-Sequence (PLL-Driven)/1 -> Gain2/1
  Gain2/1 -> Divide/1, V_grid_rms_posSeq_SI/1
  Gain3/1 -> Divide/2, I_grid_rms_posSeq_SI/1
  Gain4/1 -> V_breaker_rms_posSeq_SI/1
  Divide/1 -> Gain5/1
  Positive-Sequence (PLL-Driven)2/2 -> Gain7/1
  Gain5/1 -> Product1/1, Product/1  "S_grid_SI"
  Positive-Sequence (PLL-Driven)/2 -> Gain1/1, Add/1
  Positive-Sequence (PLL-Driven)1/2 -> Add/2
  Add/1 -> Gain6/1
  Gain6/1 -> Trigonometric Function1/1, Trigonometric Function/1  "phi_grid"
  Product1/1 -> Q_grid_SI/1
  Product/1 -> P_grid_SI/1
  Trigonometric Function/1 -> Product/2
  Trigonometric Function1/1 -> Product1/2
  PLL (3ph)/1 -> Positive-Sequence (PLL-Driven)2/1, f_grid_PLL_SI/1, Positive-Sequence (PLL-Driven)/1, Positive-Sequence (PLL-Driven)1/1
  PLL (3ph)/2 -> Positive-Sequence (PLL-Driven)/2, Positive-Sequence (PLL-Driven)2/2, Positive-Sequence (PLL-Driven)1/2
  Gain1/1 -> V_grid_phase_posSeq_SI/1
  Gain7/1 -> V_breaker_phase_posSeq_SI/1

== system Model_DG_CHP_Plant_Simscape/CHP Plant Simscape (SG based)/SI_pu_Transformation/SG_Measurements_To_SI ==
  m_pu : Inport
  Bus Creator : BusCreator  Inputs=2
  Bus Selector : BusSelector  OutputSignals=Rotor velocity (pu)
  Gain : Gain  Gain=f_n
  Gain1 : Gain  Gain=(2*pi)/nPolePairs
  m_SI : Outport
  wires:
  m_pu/1 -> Bus Selector/1
  Bus Creator/1 -> m_SI/1
  Bus Selector/1 -> Gain/1  "<Rotor velocity (pu)>"
  Gain/1 -> Bus Creator/2, Gain1/1  "Frequency (Hz)"
  Gain1/1 -> Bus Creator/1  "Roter velocity (rad/s)"

== system Model_DG_CHP_Plant_Simscape/CHP Plant Simscape (SG based)/SG_Control/Exciter/AC1A ==
  Vref : Inport
  Vt : Inport  Port=2
  It : Inport  Port=3
  Ifd : Inport  Port=4
  Vstab : Inport  Port=5
  AC1A : spsAC1AExcitationSystemLib/AC1A Excitation System  Tr=20e-3  KaTa=[400 0.02]  VAminmax=[-14.5 14.5]  VRminmax=[-5.43 6.03]  KfTf=[0.03 1.0]  TbTc=[0 0]  KeTe=[1.0 0.80]  Ve12=[4.18 3.14]  SeVe12=[0.10 0.03]  Kd=0.38  Kc=0.20  v0=[0.000416667,0.000461832]*0  TsBlock=-2
  term3 : Terminator
  Efd : Outport  VectorParamsAs1DForOutWhenUnconnected=off
  wires:
  Vref/1 -> AC1A/1
  Vt/1 -> AC1A/2
  Ifd/1 -> AC1A/3
  Vstab/1 -> AC1A/4
  AC1A/1 -> Efd/1
  It/1 -> term3/1

== system Model_DG_CHP_Plant_Simscape/CHP Plant Simscape (SG based)/SG_Control/Exciter/AC4A ==
  Vref : Inport
  Vt : Inport  Port=2
  It : Inport  Port=3
  Ifd : Inport  Port=4
  Vstab : Inport  Port=5
  AC4A : sps_avr/AC4A Excitation System  Tr=20e-3  KaTa=[200 0.015]  VIminmax=[-10 10]  VRminmax=[-4.53 5.64]  TbTc=[10 1.0]  Kc=0  v0=[1,1.42734]  TsBlock=-2
  term3 : Terminator
  Efd : Outport  VectorParamsAs1DForOutWhenUnconnected=off
  wires:
  Vref/1 -> AC4A/1
  Vt/1 -> AC4A/2
  Ifd/1 -> AC4A/3
  Vstab/1 -> AC4A/4
  AC4A/1 -> Efd/1
  It/1 -> term3/1

== system Model_DG_CHP_Plant_Simscape/CHP Plant Simscape (SG based)/SG_Control/Exciter/AC5A ==
  Vref : Inport
  Vt : Inport  Port=2
  It : Inport  Port=3
  Ifd : Inport  Port=4
  Vstab : Inport  Port=5
  AC5A : sps_avr/AC5A Excitation System  Tr=20e-3  KaTa=[100 0.02]  VRminmax=[-7.3 7.3]  KfTf=[0.03 1 0 0]  KeTe=[1.0 0.8]  Efd12=[5.6 0.75*5.6]  SeEfd12=[0.86 0.5]  v0=[1,1.42734]  TsBlock=-2
  term3 : Terminator
  term4 : Terminator
  Efd : Outport  VectorParamsAs1DForOutWhenUnconnected=off
  wires:
  Vref/1 -> AC5A/1
  Vt/1 -> AC5A/2
  Vstab/1 -> AC5A/3
  AC5A/1 -> Efd/1
  It/1 -> term3/1
  Ifd/1 -> term4/1

== system Model_DG_CHP_Plant_Simscape/CHP Plant Simscape (SG based)/SG_Control/Exciter/DC1A ==
  Vref : Inport
  Vt : Inport  Port=2
  It : Inport  Port=3
  Ifd : Inport  Port=4
  Vstab : Inport  Port=5
  DC1A : sps_avr/DC1A Excitation System  Tr=20e-3  KaTa=[46 0.06]  VRminmax=[-0.9 1.0]  KfTf=[0.1 1]  TbTc=[0 0]  KeTe=[0.05 0.46]  Efd12=[3.1 2.3]  SeEfd12=[0.33 0.10]  v0=[1,1.42734]  TsBlock=-2
  term3 : Terminator
  term4 : Terminator
  Efd : Outport  VectorParamsAs1DForOutWhenUnconnected=off
  wires:
  Vref/1 -> DC1A/1
  Vt/1 -> DC1A/2
  Vstab/1 -> DC1A/3
  DC1A/1 -> Efd/1
  It/1 -> term3/1
  Ifd/1 -> term4/1
